simulink model "B5_Signal"  (R2022b)
settings: Solver=FixedStepDiscrete  StartTime=0.0  StopTime=20  FixedStep=Ts  RelTol=1e-3
values from neighbouring files (symbols this model uses):
  Ts = 0.01    [build_B2_AutoHeadlamp.m]    (also in build_B3_AHB.m)
undefined symbols (not defined in the file or in its folder): A_ESS_OFF, A_ESS_ON, F_BLINK, F_ESS, F_HYPER, N_COMFORT, T_SHORT, V_ESS, V_RESUME
settings Model: Creator=LENOVO  LastModifiedBy=LENOVO

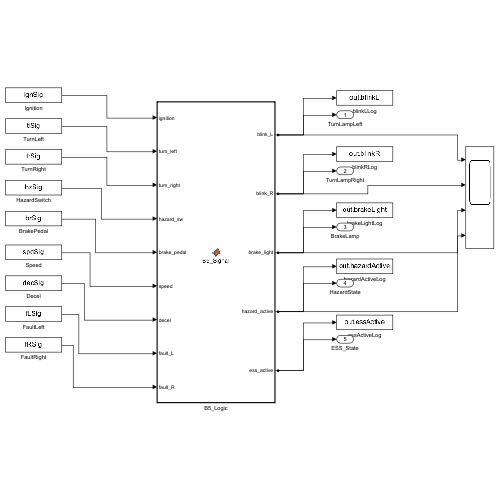
[thumbnail: Simulink's stored preview of the top-level diagram]
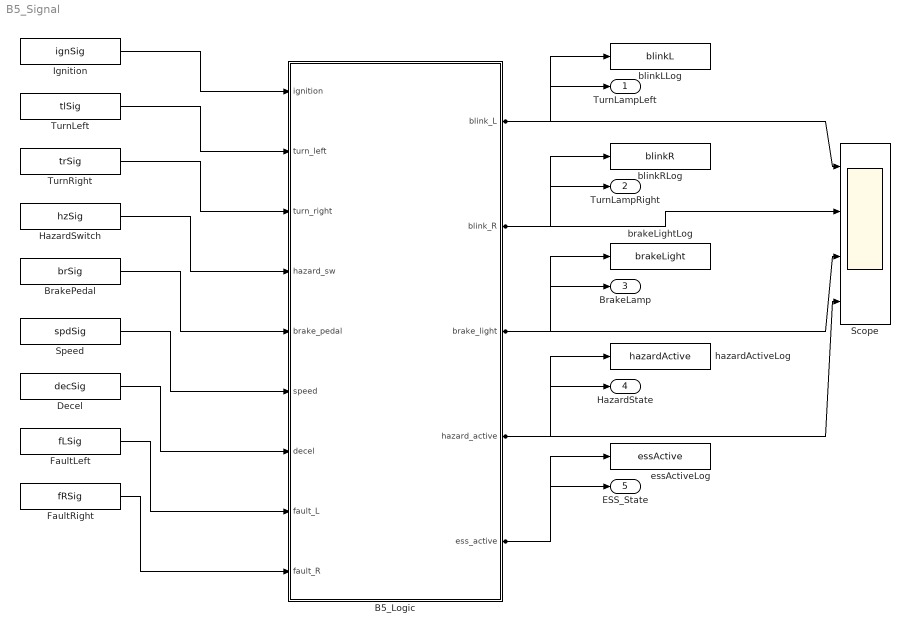
== system B5_Signal ==
  B5_Logic : MATLAB Function  TreatAsAtomicUnit=on
  BrakePedal : FromWorkspace  VariableName=brSig  SampleTime=Ts  Interpolate=off  OutputAfterFinalValue=Holding final value
  Decel : FromWorkspace  VariableName=decSig  SampleTime=Ts  OutputAfterFinalValue=Holding final value
  FaultLeft : FromWorkspace  VariableName=fLSig  SampleTime=Ts  Interpolate=off  OutputAfterFinalValue=Holding final value
  FaultRight : FromWorkspace  VariableName=fRSig  SampleTime=Ts  Interpolate=off  OutputAfterFinalValue=Holding final value
  HazardSwitch : FromWorkspace  VariableName=hzSig  SampleTime=Ts  Interpolate=off  OutputAfterFinalValue=Holding final value
  Ignition : FromWorkspace  VariableName=ignSig  SampleTime=Ts  Interpolate=off  OutputAfterFinalValue=Holding final value
  Scope : Scope  NumInputPorts=4
  Speed : FromWorkspace  VariableName=spdSig  SampleTime=Ts  OutputAfterFinalValue=Holding final value
  TurnLeft : FromWorkspace  VariableName=tlSig  SampleTime=Ts  Interpolate=off  OutputAfterFinalValue=Holding final value
  TurnRight : FromWorkspace  VariableName=trSig  SampleTime=Ts  Interpolate=off  OutputAfterFinalValue=Holding final value
  blinkLLog : ToWorkspace  VariableName=blinkL  SaveFormat=Timeseries  SampleTime=-1
  blinkRLog : ToWorkspace  VariableName=blinkR  SaveFormat=Timeseries  SampleTime=-1
  brakeLightLog : ToWorkspace  VariableName=brakeLight  SaveFormat=Timeseries  SampleTime=-1
  essActiveLog : ToWorkspace  VariableName=essActive  SaveFormat=Timeseries  SampleTime=-1
  hazardActiveLog : ToWorkspace  VariableName=hazardActive  SaveFormat=Timeseries  SampleTime=-1
  TurnLampLeft : Outport
  TurnLampRight : Outport  Port=2
  BrakeLamp : Outport  Port=3
  HazardState : Outport  Port=4
  ESS_State : Outport  Port=5
  wires:
  Ignition/1 -> B5_Logic/1(ignition)
  TurnLeft/1 -> B5_Logic/2(turn_left)
  TurnRight/1 -> B5_Logic/3(turn_right)
  HazardSwitch/1 -> B5_Logic/4(hazard_sw)
  BrakePedal/1 -> B5_Logic/5(brake_pedal)
  Speed/1 -> B5_Logic/6(speed)
  Decel/1 -> B5_Logic/7(decel)
  FaultLeft/1 -> B5_Logic/8(fault_L)
  FaultRight/1 -> B5_Logic/9(fault_R)
  B5_Logic/1(blink_L) -> blinkLLog/1, TurnLampLeft/1, Scope/1
  B5_Logic/2(blink_R) -> blinkRLog/1, TurnLampRight/1, Scope/2
  B5_Logic/3(brake_light) -> brakeLightLog/1, BrakeLamp/1, Scope/3
  B5_Logic/4(hazard_active) -> hazardActiveLog/1, HazardState/1, Scope/4
  B5_Logic/5(ess_active) -> essActiveLog/1, ESS_State/1

== matlab function B5_Signal/B5_Logic ==
  data: ignition input; blink_L output; turn_left input; turn_right input; hazard_sw input; brake_pedal input; speed input; decel input; fault_L input; fault_R input; blink_R output; brake_light output; hazard_active output; ess_active output; Ts parameter; F_BLINK parameter; F_HYPER parameter; T_SHORT parameter; N_COMFORT parameter; A_ESS_ON parameter; A_ESS_OFF parameter; V_ESS parameter; F_ESS parameter; V_RESUME parameter
function [blink_L, blink_R, brake_light, hazard_active, ess_active] = B5_Signal(ignition, turn_left, turn_right, hazard_sw, brake_pedal, speed, decel, fault_L, fault_R, Ts, F_BLINK, F_HYPER, T_SHORT, N_COMFORT, A_ESS_ON, A_ESS_OFF, V_ESS, F_ESS, V_RESUME)
%#codegen
% B5 - Clignotants, feux de detresse, feux stop et signal de freinage d'urgence (ESS)
% decel : deceleration longitudinale [m/s2], positive quand le vehicule freine
persistent init tside comfort press_t prevL prevR prev_req ph cyc ess ph_ess ess_seen auto_haz
if isempty(init)
    init = true; tside = 0; comfort = false; press_t = 0; prevL = false; prevR = false;
    prev_req = 0; ph = 0; cyc = 0; ess = false; ph_ess = 0; ess_seen = false; auto_haz = false;
end

% ---------- 1) Signal de freinage d'urgence ESS (REQ-LSC-20)
if ~ess && brake_pedal && decel > A_ESS_ON && speed > V_ESS
    ess = true; ph_ess = 0; ess_seen = true;          % freinage d'urgence detecte
elseif ess && (decel < A_ESS_OFF || ~brake_pedal)
    ess = false;                                       % fin du freinage d'urgence
end

% ---------- 2) Feux de detresse automatiques apres arret d'urgence (REQ-LSC-21)
if ess_seen && speed < 0.5
    auto_haz = true; ess_seen = false;
end
if auto_haz && speed > V_RESUME
    auto_haz = false;                                  % le vehicule repart
end
hazard = hazard_sw || auto_haz;

% ---------- 3) Demande de clignotement : 0 aucun, 1 gauche, 2 droite, 3 detresse
if hazard
    req = 3;                                           % detresse prioritaire, meme contact coupe (REQ-LSC-18)
    tside = 0; comfort = false;
elseif ignition
    if turn_left && ~prevL                             % debut d'appui a gauche
        tside = 1; press_t = 0; comfort = false;
    elseif turn_right && ~prevR                        % debut d'appui a droite
        tside = 2; press_t = 0; comfort = false;
    end
    if (tside == 1 && turn_left) || (tside == 2 && turn_right)
        press_t = press_t + Ts;                        % duree d'appui
    end
    if (tside == 1 && ~turn_left && prevL) || (tside == 2 && ~turn_right && prevR)
        if press_t < T_SHORT
            comfort = true;                            % impulsion courte : mode autoroute (REQ-LSC-17)
        else
            tside = 0;                                 % levier relache : arret
        end
    end
    if comfort && cyc >= N_COMFORT
        tside = 0; comfort = false;                    % 3 cycles effectues
    end
    req = tside;
else
    req = 0; tside = 0; comfort = false;
end
prevL = turn_left; prevR = turn_right;

% ---------- 4) Generateur de clignotement (REQ-LSC-16, hyper-clignotement REQ-LSC-23)
if (req == 1 && fault_L) || (req == 2 && fault_R) || (req == 3 && (fault_L || fault_R))
    period = 1 / F_HYPER;                              % lampe grillee : frequence doublee
else
    period = 1 / F_BLINK;
end
if req ~= prev_req
    ph = 0; cyc = 0;                                   % nouvelle demande : on repart d'un flash allume
end
prev_req = req;
on = false;
if req > 0
    on = ph < period / 2;                              % rapport cyclique 50 %
    ph = ph + Ts;
    if ph >= period - 1e-9
        ph = ph - period; cyc = cyc + 1;               % un cycle complet
    end
end
blink_L = on && (req == 1 || req == 3);
blink_R = on && (req == 2 || req == 3);

% ---------- 5) Feux stop (REQ-LSC-19) et clignotement ESS
if ess
    brake_light = ph_ess < 0.5 / F_ESS;
    ph_ess = ph_ess + Ts;
    if ph_ess >= 1 / F_ESS - 1e-9, ph_ess = ph_ess - 1 / F_ESS; end
else
    brake_light = brake_pedal;                         % allumage direct a l'appui
end
hazard_active = hazard;
ess_active = ess;
